simulink model "uav"  (R2013a)
settings: Solver=ode45  StartTime=0.0  StopTime=50  RelTol=1e-3
values from neighbouring files (symbols this model uses):
  g = S.g; else g = 9.81; warning('g not found, using 9.81'); end    [LQR_implementation.m]    (also in allvars.mat = 9.81; lqr_gains.mat = 9.81)
  I = diag([Ixx_local Iyy_local Izz_local])    [LQR_implementation.m]    (also in allvars.mat = 0.2)
  I1 = 1.25    [allvars.mat]
  I2 = 1.25    [allvars.mat]
  I3 = 2.5    [allvars.mat]
  K1 = 0.01    [allvars.mat]
  K2 = 0.01    [allvars.mat]
  K3 = 0.01    [allvars.mat]
  K4 = 0.012    [allvars.mat]
  K5 = 0.012    [allvars.mat]
  K6 = 0.012    [allvars.mat]
  m = 2    [allvars.mat]    (also in lqr_gains.mat)
libraries: simulink x4
settings Model: Creator=MUKUL GAUR  LastModifiedBy=Himanshu

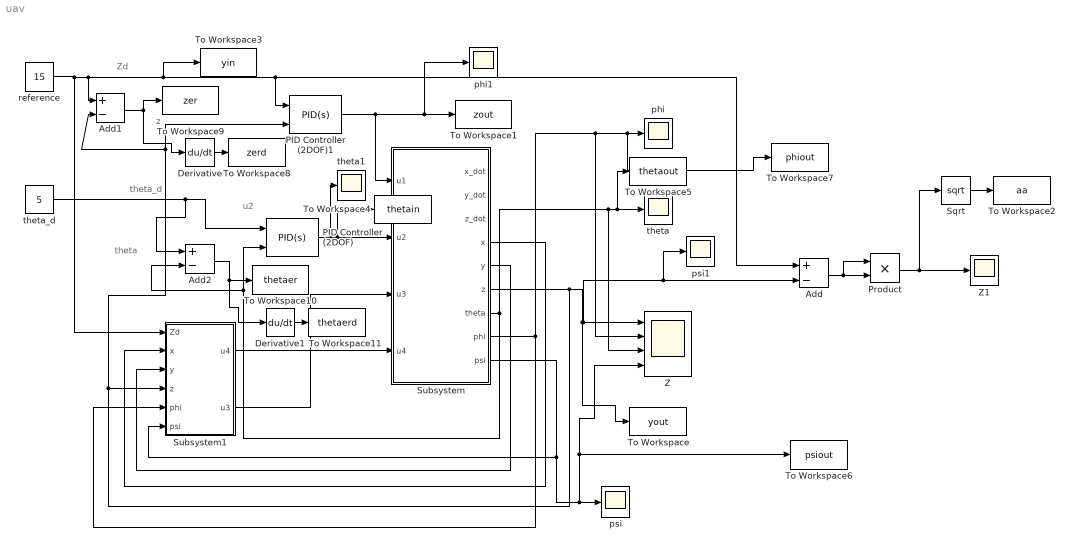
== system uav ==
  note: Zd
  note: z
  note: u2
  note: theta
  note: theta_d
  Add : Sum  Inputs=+-
  Add1 : Sum  Inputs=+-
  Add2 : Sum  Inputs=+-
  Derivative : Derivative
  Derivative1 : Derivative
  PID Controller (2DOF) : simulink/Continuous/PID Controller (2DOF)  Controller=PID  TimeDomain=Continuous-time  SampleTime=1  IntegratorMethod=Forward Euler  FilterMethod=Forward Euler  Form=Parallel  P=1.37615732997435e-04  I=25.5863973899387e-05  D=10.357891563648134  N=1.925490537332276  b=1  c=1  InitialConditionSource=internal  InitialConditionForIntegrator=0  InitialConditionForFilter=0  ExternalReset=none  LimitOutput=off  UpperSaturationLimit=inf  LowerSaturationLimit=-inf  LinearizeAsGain=on  AntiWindupMode=none  Kb=1  TrackingMode=off  Kt=1  PParamMin=[]  PParamMax=[]  IParamMin=[]  IParamMax=[]  DParamMin=[]  DParamMax=[]  NParamMin=[]  NParamMax=[]  bParamMin=[]  bParamMax=[]  cParamMin=[]  cParamMax=[]  KbParamMin=[]  KbParamMax=[]  KtParamMin=[]  KtParamMax=[]  POutMin=[]  POutMax=[]  IOutMin=[]  IOutMax=[]  DOutMin=[]  DOutMax=[]  NOutMin=[]  NOutMax=[]  bOutMin=[]  bOutMax=[]  cOutMin=[]  cOutMax=[]  KbOutMin=[]  KbOutMax=[]  KtOutMin=[]  KtOutMax=[]  IntegratorOutMin=[]  IntegratorOutMax=[]  FilterOutMin=[]  FilterOutMax=[]  SumOutMin=[]  SumOutMax=[]  Sum1OutMin=[]  Sum1OutMax=[]  Sum2OutMin=[]  Sum2OutMax=[]  Sum3OutMin=[]  Sum3OutMax=[]  SumI1OutMin=[]  SumI1OutMax=[]  SumI2OutMin=[]  SumI2OutMax=[]  SumI3OutMin=[]  SumI3OutMax=[]  SumDOutMin=[]  SumDOutMax=[]  SaturationOutMin=[]  SaturationOutMax=[]  IntegratorContinuousStateAttributes=''  IntegratorStateMustResolveToSignalObject=off  IntegratorRTWStateStorageClass=Auto  FilterContinuousStateAttributes=''  FilterStateMustResolveToSignalObject=off  FilterRTWStateStorageClass=Auto
  PID Controller (2DOF)1 : simulink/Continuous/PID Controller (2DOF)  Controller=PID  TimeDomain=Continuous-time  SampleTime=1  IntegratorMethod=Forward Euler  FilterMethod=Forward Euler  Form=Parallel  P=2.58553  I=300.999406  D=80.9375  N=8.889996  b=1  c=1  InitialConditionSource=internal  InitialConditionForIntegrator=0  InitialConditionForFilter=0  ExternalReset=none  LimitOutput=off  UpperSaturationLimit=inf  LowerSaturationLimit=-inf  LinearizeAsGain=on  AntiWindupMode=none  Kb=1  TrackingMode=off  Kt=1  PParamMin=[]  PParamMax=[]  IParamMin=[]  IParamMax=[]  DParamMin=[]  DParamMax=[]  NParamMin=[]  NParamMax=[]  bParamMin=[]  bParamMax=[]  cParamMin=[]  cParamMax=[]  KbParamMin=[]  KbParamMax=[]  KtParamMin=[]  KtParamMax=[]  POutMin=[]  POutMax=[]  IOutMin=[]  IOutMax=[]  DOutMin=[]  DOutMax=[]  NOutMin=[]  NOutMax=[]  bOutMin=[]  bOutMax=[]  cOutMin=[]  cOutMax=[]  KbOutMin=[]  KbOutMax=[]  KtOutMin=[]  KtOutMax=[]  IntegratorOutMin=[]  IntegratorOutMax=[]  FilterOutMin=[]  FilterOutMax=[]  SumOutMin=[]  SumOutMax=[]  Sum1OutMin=[]  Sum1OutMax=[]  Sum2OutMin=[]  Sum2OutMax=[]  Sum3OutMin=[]  Sum3OutMax=[]  SumI1OutMin=[]  SumI1OutMax=[]  SumI2OutMin=[]  SumI2OutMax=[]  SumI3OutMin=[]  SumI3OutMax=[]  SumDOutMin=[]  SumDOutMax=[]  SaturationOutMin=[]  SaturationOutMax=[]  IntegratorContinuousStateAttributes=''  IntegratorStateMustResolveToSignalObject=off  IntegratorRTWStateStorageClass=Auto  FilterContinuousStateAttributes=''  FilterStateMustResolveToSignalObject=off  FilterRTWStateStorageClass=Auto
  Product : Product
  Sqrt : Sqrt  SaturateOnIntegerOverflow=on
  Subsystem : Subsystem
  Subsystem1 : Subsystem
  To Workspace : ToWorkspace  VariableName=yout  SampleTime=-1
  To Workspace1 : ToWorkspace  VariableName=zout  SampleTime=-1
  To Workspace10 : ToWorkspace  VariableName=thetaer  SampleTime=-1
  To Workspace11 : ToWorkspace  VariableName=thetaerd  SampleTime=-1
  To Workspace2 : ToWorkspace  VariableName=aa  SampleTime=-1  SaveFormat=Structure
  To Workspace3 : ToWorkspace  VariableName=yin  SampleTime=-1
  To Workspace4 : ToWorkspace  VariableName=thetain  SampleTime=-1
  To Workspace5 : ToWorkspace  VariableName=thetaout  SampleTime=-1
  To Workspace6 : ToWorkspace  VariableName=psiout  SampleTime=-1
  To Workspace7 : ToWorkspace  VariableName=phiout  SampleTime=-1
  To Workspace8 : ToWorkspace  VariableName=zerd  SampleTime=-1
  To Workspace9 : ToWorkspace  VariableName=zer  SampleTime=-1
  Z : Scope  NumInputPorts=4
      settings: YMin=8~-5~-5~-5  YMax=11.5~5~5~5  SaveName=ScopeData2
  Z1 : Scope
      settings: YMin=8  YMax=11.5  SaveName=ScopeData4
  phi : Scope
      settings: YMin=264.654  YMax=292.512
  phi1 : Scope
      settings: YMin=264.654  YMax=292.512  SaveName=ScopeData8
  psi : Scope
      settings: TimeRange=50  YMin=-4e+21  YMax=-1.5e+21  SaveName=ScopeData3
  psi1 : Scope
      settings: TimeRange=50  YMin=-4e+21  YMax=-1.5e+21  SaveName=ScopeData9
  reference : Constant  Value=15
  theta : Scope
      settings: YMin=19398.1  YMax=21440.1
  theta1 : Scope
      settings: YMin=19398.1  YMax=21440.1  SaveName=ScopeData7
  theta_d : Constant  Value=5
  wires:
  theta_d/1 -> Add2/1, PID Controller (2DOF)/1
  Subsystem/4(x) -> Subsystem1/2(x)
  Subsystem/5(y) -> Subsystem1/3(y)
  Subsystem/8(phi) -> Subsystem1/5(phi), Z/2, To Workspace7/1, phi/1
  Subsystem/9(psi) -> Subsystem1/6(psi), To Workspace6/1, Z/4, psi/1
  Subsystem1/2(u3) -> Subsystem/3(u3)
  Subsystem1/1(u4) -> Subsystem/4(u4)
  PID Controller (2DOF)/1 -> theta1/1, To Workspace4/1, Subsystem/2(u2)
  PID Controller (2DOF)1/1 -> phi1/1, To Workspace1/1, Subsystem/1(u1)
  Subsystem/6(z) -> PID Controller (2DOF)1/2, Add1/2, Subsystem1/4(z), To Workspace/1, psi1/1, Add/2, Z/1
  reference/1 -> Subsystem1/1(Zd), Add1/1, To Workspace3/1, Add/1, PID Controller (2DOF)1/1
  Add/1 -> Product/1, Product/2
  Product/1 -> Sqrt/1, Z1/1
  Sqrt/1 -> To Workspace2/1
  Add1/1 -> Derivative/1, To Workspace9/1
  Derivative/1 -> To Workspace8/1
  Subsystem/7(theta) -> Add2/2, PID Controller (2DOF)/2, Z/3, To Workspace5/1, theta/1
  Add2/1 -> Derivative1/1, To Workspace10/1
  Derivative1/1 -> To Workspace11/1

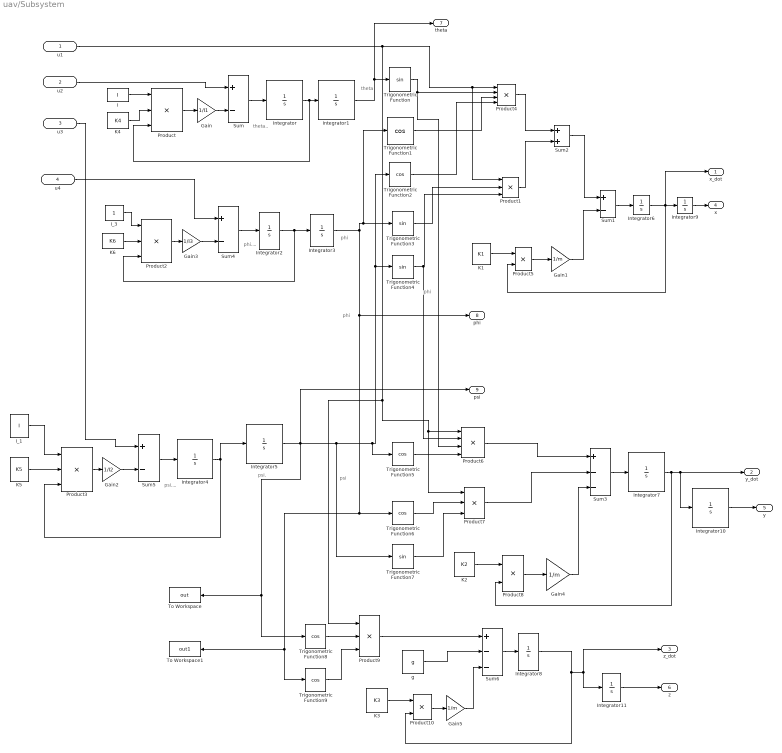
== system uav/Subsystem ==
  note: phi
  note: phi
  note: psi
  note: phi
  note: theta
  note: theta..
  note: phi....
  note: psi.
  note: psi....
  u1 : Inport
  u2 : Inport  Port=2
  u3 : Inport  Port=3
  u4 : Inport  Port=4
  Gain : Gain  Gain=1/I1
  Gain1 : Gain  Gain=1/m
  Gain2 : Gain  Gain=1/I2
  Gain3 : Gain  Gain=1/I3
  Gain4 : Gain  Gain=1/m
  Gain5 : Gain  Gain=1/m
  I : Constant  Value=I
  I_1 : Constant  Value=I
  I_3 : Constant
  Integrator{,1..11} (12 alike) : Integrator
  K1 : Constant  Value=K1
  K2 : Constant  Value=K2
  K3 : Constant  Value=K3
  K4 : Constant  Value=K4
  K5 : Constant  Value=K5
  K6 : Constant  Value=K6
  Product{,1..3,7,9} (6 alike) : Product  Inputs=3
  Product10 : Product
  Product4 : Product  Inputs=4
  Product5 : Product
  Product6 : Product  Inputs=4
  Product8 : Product
  Sum{,1,4..5} (4 alike) : Sum  Inputs=+-
  Sum2 : Sum
  Sum3 : Sum  Inputs=+--
  Sum6 : Sum  Inputs=+--
  To Workspace : ToWorkspace  VariableName=out  SampleTime=-1
  To Workspace1 : ToWorkspace  VariableName=out1  SampleTime=-1
  Trigonometric Function{,3..4,7} (4 alike) : Trigonometry
  Trigonometric Function{1..2,5..6,8..9} (6 alike) : Trigonometry  Operator=cos
  g : Constant  Value=g
  x_dot : Outport
  y_dot : Outport  Port=2
  z_dot : Outport  Port=3
  x : Outport  Port=4
  y : Outport  Port=5
  z : Outport  Port=6
  theta : Outport  Port=7
  phi : Outport  Port=8
  psi : Outport  Port=9
  wires:
  Integrator5/1 -> Trigonometric Function8/1, To Workspace/1, Trigonometric Function7/1, Trigonometric Function5/1, Trigonometric Function4/1, Trigonometric Function2/1, psi/1
  g/1 -> Sum6/2
  Sum6/1 -> Integrator8/1
  Integrator8/1 -> z_dot/1, Integrator11/1, Product10/2
  K3/1 -> Product10/1
  Product10/1 -> Gain5/1
  Gain5/1 -> Sum6/3
  Integrator9/1 -> x/1
  Integrator10/1 -> y/1
  Integrator11/1 -> z/1
  Trigonometric Function2/1 -> Product4/4
  Trigonometric Function1/1 -> Product4/3
  u1/1 -> Product1/1, Product4/1, Product9/1, Product7/1, Product6/1
  K5/1 -> Product3/2
  Product3/1 -> Gain2/1
  Sum5/1 -> Integrator4/1
  Integrator4/1 -> Product3/3, Integrator5/1
  I_1/1 -> Product3/1
  Trigonometric Function8/1 -> Product9/2
  Trigonometric Function9/1 -> Product9/3
  Sum1/1 -> Integrator6/1
  K2/1 -> Product8/1
  Sum3/1 -> Integrator7/1
  Integrator7/1 -> y_dot/1, Integrator10/1, Product8/2
  Gain1/1 -> Sum1/2
  Product8/1 -> Gain4/1
  Gain4/1 -> Sum3/3
  Trigonometric Function4/1 -> Product6/2, Product1/3
  Trigonometric Function3/1 -> Product1/2
  Trigonometric Function/1 -> Product6/3, Product4/2
  Trigonometric Function5/1 -> Product6/4
  Product4/1 -> Sum2/1
  Product1/1 -> Sum2/2
  Trigonometric Function6/1 -> Product7/2
  Trigonometric Function7/1 -> Product7/3
  Sum/1 -> Integrator/1
  Product/1 -> Gain/1
  Gain/1 -> Sum/2
  K6/1 -> Product2/2
  Gain3/1 -> Sum4/2
  Integrator2/1 -> Product2/3, Integrator3/1
  Sum4/1 -> Integrator2/1
  Product2/1 -> Gain3/1
  I/1 -> Product/1
  K4/1 -> Product/2
  Integrator/1 -> Product/3, Integrator1/1
  u2/1 -> Sum/1
  Integrator6/1 -> Integrator9/1, x_dot/1, Product5/2
  K1/1 -> Product5/1
  Product5/1 -> Gain1/1
  Integrator1/1 -> theta/1, Trigonometric Function/1
  u4/1 -> Sum4/1
  u3/1 -> Sum5/1
  Gain2/1 -> Sum5/2
  Sum2/1 -> Sum1/1
  Product7/1 -> Sum3/2
  Product6/1 -> Sum3/1
  Product9/1 -> Sum6/1
  I_3/1 -> Product2/1
  Integrator3/1 -> Trigonometric Function3/1, Trigonometric Function1/1, phi/1, Trigonometric Function6/1, Trigonometric Function9/1, To Workspace1/1

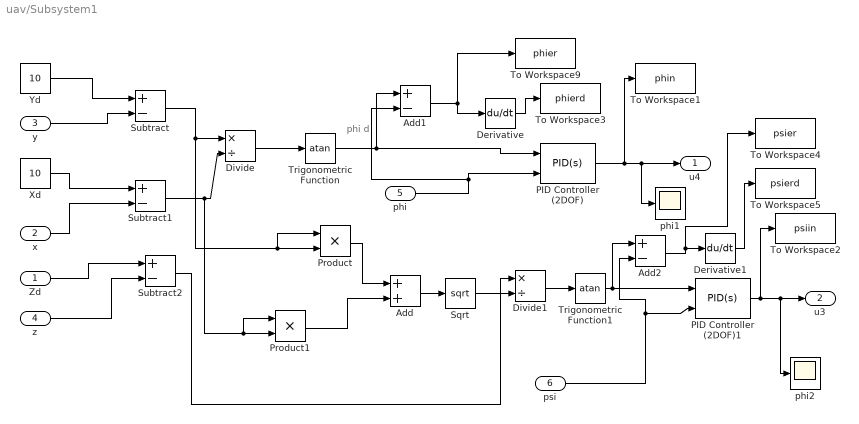
== system uav/Subsystem1 ==
  note: phi d
  Zd : Inport
  x : Inport  Port=2
  y : Inport  Port=3
  z : Inport  Port=4
  phi : Inport  Port=5
  psi : Inport  Port=6
  Add : Sum
  Add1 : Sum  Inputs=+-
  Add2 : Sum  Inputs=+-
  Derivative : Derivative
  Derivative1 : Derivative
  Divide : Product  Inputs=*/
  Divide1 : Product  Inputs=*/
  PID Controller (2DOF) : simulink/Continuous/PID Controller (2DOF)  Controller=PID  TimeDomain=Continuous-time  SampleTime=1  IntegratorMethod=Forward Euler  FilterMethod=Forward Euler  Form=Parallel  P=9.0398509833123405  I=10.4787459217742e-07  D=120.894728909120335  N=7.231372634333069  b=1  c=1  InitialConditionSource=internal  InitialConditionForIntegrator=0  InitialConditionForFilter=0  ExternalReset=none  LimitOutput=off  UpperSaturationLimit=inf  LowerSaturationLimit=-inf  LinearizeAsGain=on  AntiWindupMode=none  Kb=1  TrackingMode=off  Kt=1  PParamMin=[]  PParamMax=[]  IParamMin=[]  IParamMax=[]  DParamMin=[]  DParamMax=[]  NParamMin=[]  NParamMax=[]  bParamMin=[]  bParamMax=[]  cParamMin=[]  cParamMax=[]  KbParamMin=[]  KbParamMax=[]  KtParamMin=[]  KtParamMax=[]  POutMin=[]  POutMax=[]  IOutMin=[]  IOutMax=[]  DOutMin=[]  DOutMax=[]  NOutMin=[]  NOutMax=[]  bOutMin=[]  bOutMax=[]  cOutMin=[]  cOutMax=[]  KbOutMin=[]  KbOutMax=[]  KtOutMin=[]  KtOutMax=[]  IntegratorOutMin=[]  IntegratorOutMax=[]  FilterOutMin=[]  FilterOutMax=[]  SumOutMin=[]  SumOutMax=[]  Sum1OutMin=[]  Sum1OutMax=[]  Sum2OutMin=[]  Sum2OutMax=[]  Sum3OutMin=[]  Sum3OutMax=[]  SumI1OutMin=[]  SumI1OutMax=[]  SumI2OutMin=[]  SumI2OutMax=[]  SumI3OutMin=[]  SumI3OutMax=[]  SumDOutMin=[]  SumDOutMax=[]  SaturationOutMin=[]  SaturationOutMax=[]  IntegratorContinuousStateAttributes=''  IntegratorStateMustResolveToSignalObject=off  IntegratorRTWStateStorageClass=Auto  FilterContinuousStateAttributes=''  FilterStateMustResolveToSignalObject=off  FilterRTWStateStorageClass=Auto
  PID Controller (2DOF)1 : simulink/Continuous/PID Controller (2DOF)  Controller=PID  TimeDomain=Continuous-time  SampleTime=1  IntegratorMethod=Forward Euler  FilterMethod=Forward Euler  Form=Parallel  P=4.37615732997435e-05  I=4.5863973899387e-08  D=10.0357891563648134  N=3.0925490537332276  b=1  c=1  InitialConditionSource=internal  InitialConditionForIntegrator=0  InitialConditionForFilter=0  ExternalReset=none  LimitOutput=off  UpperSaturationLimit=inf  LowerSaturationLimit=-inf  LinearizeAsGain=on  AntiWindupMode=none  Kb=1  TrackingMode=off  Kt=1  PParamMin=[]  PParamMax=[]  IParamMin=[]  IParamMax=[]  DParamMin=[]  DParamMax=[]  NParamMin=[]  NParamMax=[]  bParamMin=[]  bParamMax=[]  cParamMin=[]  cParamMax=[]  KbParamMin=[]  KbParamMax=[]  KtParamMin=[]  KtParamMax=[]  POutMin=[]  POutMax=[]  IOutMin=[]  IOutMax=[]  DOutMin=[]  DOutMax=[]  NOutMin=[]  NOutMax=[]  bOutMin=[]  bOutMax=[]  cOutMin=[]  cOutMax=[]  KbOutMin=[]  KbOutMax=[]  KtOutMin=[]  KtOutMax=[]  IntegratorOutMin=[]  IntegratorOutMax=[]  FilterOutMin=[]  FilterOutMax=[]  SumOutMin=[]  SumOutMax=[]  Sum1OutMin=[]  Sum1OutMax=[]  Sum2OutMin=[]  Sum2OutMax=[]  Sum3OutMin=[]  Sum3OutMax=[]  SumI1OutMin=[]  SumI1OutMax=[]  SumI2OutMin=[]  SumI2OutMax=[]  SumI3OutMin=[]  SumI3OutMax=[]  SumDOutMin=[]  SumDOutMax=[]  SaturationOutMin=[]  SaturationOutMax=[]  IntegratorContinuousStateAttributes=''  IntegratorStateMustResolveToSignalObject=off  IntegratorRTWStateStorageClass=Auto  FilterContinuousStateAttributes=''  FilterStateMustResolveToSignalObject=off  FilterRTWStateStorageClass=Auto
  Product : Product
  Product1 : Product
  Sqrt : Sqrt  SaturateOnIntegerOverflow=on
  Subtract : Sum  Inputs=+-
  Subtract1 : Sum  Inputs=+-
  Subtract2 : Sum  Inputs=+-
  To Workspace1 : ToWorkspace  VariableName=phin  SampleTime=-1
  To Workspace2 : ToWorkspace  VariableName=psiin  SampleTime=-1
  To Workspace3 : ToWorkspace  VariableName=phierd  SampleTime=-1
  To Workspace4 : ToWorkspace  VariableName=psier  SampleTime=-1
  To Workspace5 : ToWorkspace  VariableName=psierd  SampleTime=-1
  To Workspace9 : ToWorkspace  VariableName=phier  SampleTime=-1
  Trigonometric Function : Trigonometry  Operator=atan
  Trigonometric Function1 : Trigonometry  Operator=atan
  Xd : Constant  Value=10
  Yd : Constant  Value=10
  phi1 : Scope
      settings: YMin=264.654  YMax=292.512  SaveName=ScopeData5
  phi2 : Scope
      settings: YMin=264.654  YMax=292.512  SaveName=ScopeData6
  u4 : Outport
  u3 : Outport  Port=2
  wires:
  psi/1 -> Add2/2, PID Controller (2DOF)1/2
  Subtract1/1 -> Product1/1, Product1/2, Divide/2
  Product/1 -> Add/1
  Yd/1 -> Subtract/1
  Sqrt/1 -> Divide1/2
  Divide1/1 -> Trigonometric Function1/1
  Subtract/1 -> Product/1, Product/2, Divide/1
  Divide/1 -> Trigonometric Function/1
  z/1 -> Subtract2/2
  Trigonometric Function/1 -> Add1/1, PID Controller (2DOF)/1
  Add/1 -> Sqrt/1
  Xd/1 -> Subtract1/1
  Zd/1 -> Subtract2/1
  Product1/1 -> Add/2
  y/1 -> Subtract/2
  x/1 -> Subtract1/2
  Subtract2/1 -> Divide1/1
  phi/1 -> Add1/2, PID Controller (2DOF)/2
  Trigonometric Function1/1 -> Add2/1, PID Controller (2DOF)1/1
  PID Controller (2DOF)1/1 -> To Workspace2/1, phi2/1, u3/1
  PID Controller (2DOF)/1 -> To Workspace1/1, phi1/1, u4/1
  Add1/1 -> Derivative/1, To Workspace9/1
  Derivative/1 -> To Workspace3/1
  Add2/1 -> To Workspace4/1, Derivative1/1
  Derivative1/1 -> To Workspace5/1
